simulink model "FluxObserver"  (R2026b)
settings: Solver=VariableStepAuto
undefined symbols (not defined in the file or in its folder): fluxCfg, pllCfg
libraries: AngleTracking x1
settings Model: Creator=24322  LastModifiedBy=24322

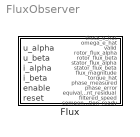
== system FluxObserver ==
  Flux : Subsystem  mask{cfg=fluxCfg, trackerCfg=pllCfg}
      mask prompts: cfg "Flux configuration"; trackerCfg "PLL configuration"

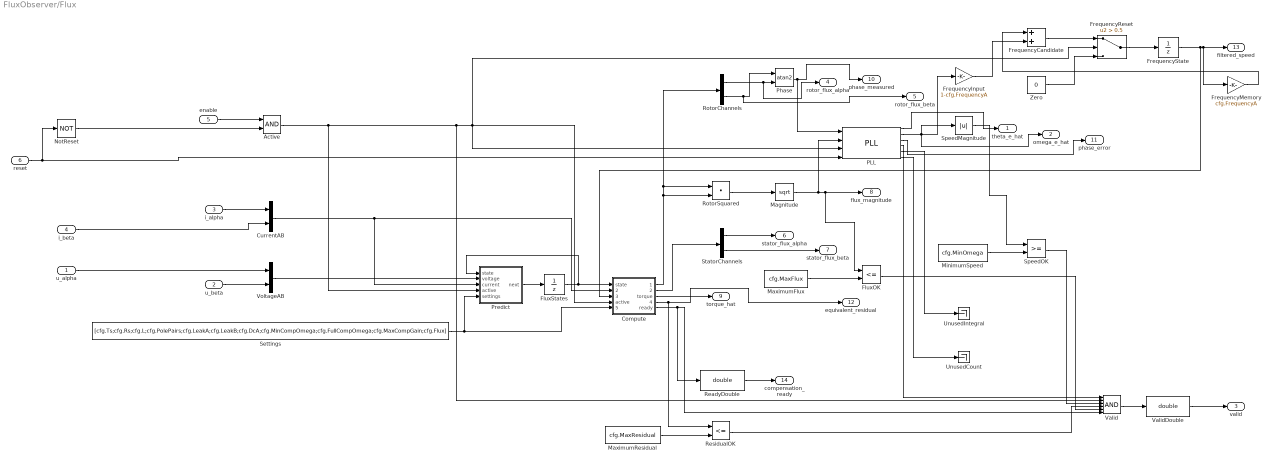
== system FluxObserver/Flux ==
  u_alpha : Inport  SampleTime=cfg.Ts
  u_beta : Inport  Port=2  SampleTime=cfg.Ts
  i_alpha : Inport  Port=3  SampleTime=cfg.Ts
  i_beta : Inport  Port=4  SampleTime=cfg.Ts
  enable : Inport  Port=5  SampleTime=cfg.Ts
  reset : Inport  Port=6  SampleTime=cfg.Ts
  Active : Logic  IconShape=distinctive  AllPortsSameDT=off  OutDataTypeStr=boolean
  Compute : MATLAB Function  TreatAsAtomicUnit=on
  CurrentAB : Mux  Inputs=2
  FluxOK : RelationalOperator  Operator=<=  OutDataTypeStr=boolean  RndMeth=Simplest  InputSameDT=off
  FluxStates : UnitDelay  InitialCondition=zeros(4,1)  SampleTime=cfg.Ts
  FrequencyCandidate : Sum
  FrequencyInput : Gain  Gain=1-cfg.FrequencyA
  FrequencyMemory : Gain  Gain=cfg.FrequencyA
  FrequencyReset : Switch  Criteria=u2 > Threshold  Threshold=0.5  SaturateOnIntegerOverflow=off  InputSameDT=off
  FrequencyState : UnitDelay  SampleTime=cfg.Ts
  Magnitude : Sqrt
  MaximumFlux : Constant  Value=cfg.MaxFlux
  MaximumResidual : Constant  Value=cfg.MaxResidual
  MinimumSpeed : Constant  Value=cfg.MinOmega
  NotReset : Logic  Operator=NOT  IconShape=distinctive  AllPortsSameDT=off  OutDataTypeStr=boolean
  PLL : AngleTracking/PLL  pllCfg=trackerCfg
  Phase : Trigonometry  Operator=atan2
  Predict : MATLAB Function  TreatAsAtomicUnit=on
  ReadyDouble : DataTypeConversion  OutDataTypeStr=double  SaturateOnIntegerOverflow=off  RndMeth=Floor
  ResidualOK : RelationalOperator  Operator=<=  OutDataTypeStr=boolean  RndMeth=Simplest  InputSameDT=off
  RotorChannels : Demux  Outputs=2
  RotorSquared : DotProduct  OutDataTypeStr=Inherit: Inherit via internal rule
  Settings : Constant  Value=[cfg.Ts;cfg.Rs;cfg.L;cfg.PolePairs;cfg.LeakA;cfg.LeakB;cfg.DcA;cfg.MinCompOmega;cfg.FullCompOmega;cfg.MaxCompGain;cfg.Flux]
  SpeedMagnitude : Abs  SaturateOnIntegerOverflow=off
  SpeedOK : RelationalOperator  OutDataTypeStr=boolean  RndMeth=Simplest  InputSameDT=off
  StatorChannels : Demux  Outputs=2
  UnusedCount : Terminator
  UnusedIntegral : Terminator
  Valid : Logic  Inputs=6  IconShape=distinctive  AllPortsSameDT=off  OutDataTypeStr=boolean
  ValidDouble : DataTypeConversion  OutDataTypeStr=double  SaturateOnIntegerOverflow=off  RndMeth=Floor
  VoltageAB : Mux  Inputs=2
  Zero : Constant  Value=0
  theta_e_hat : Outport
  omega_e_hat : Outport  Port=2
  valid : Outport  Port=3
  rotor_flux_alpha : Outport  Port=4
  rotor_flux_beta : Outport  Port=5
  stator_flux_alpha : Outport  Port=6
  stator_flux_beta : Outport  Port=7
  flux_magnitude : Outport  Port=8
  torque_hat : Outport  Port=9
  phase_measured : Outport  Port=10
  phase_error : Outport  Port=11
  equivalent_residual : Outport  Port=12
  filtered_speed : Outport  Port=13
  compensation_ready : Outport  Port=14
  wires:
  StatorChannels/2 -> stator_flux_beta/1
  StatorChannels/1 -> stator_flux_alpha/1
  PLL/6 -> UnusedCount/1
  PLL/5 -> UnusedIntegral/1
  PLL/4 -> Valid/1
  PLL/3 -> phase_error/1
  PLL/2 -> SpeedMagnitude/1, omega_e_hat/1, FrequencyInput/1
  PLL/1 -> theta_e_hat/1
  RotorChannels/1 -> Phase/2, rotor_flux_alpha/1
  RotorChannels/2 -> Phase/1, rotor_flux_beta/1
  RotorSquared/1 -> Magnitude/1
  Compute/5(ready) -> ReadyDouble/1, Valid/6
  Compute/4(residual) -> equivalent_residual/1, ResidualOK/1
  Compute/3(torque) -> torque_hat/1
  Compute/2(statorFlux) -> StatorChannels/1
  Compute/1(rotorFlux) -> RotorChannels/1, RotorSquared/1, RotorSquared/2
  Phase/1 -> PLL/1, phase_measured/1
  ReadyDouble/1 -> compensation_ready/1
  ValidDouble/1 -> valid/1
  Valid/1 -> ValidDouble/1
  FluxOK/1 -> Valid/5
  ResidualOK/1 -> Valid/4
  SpeedOK/1 -> Valid/3
  MaximumResidual/1 -> ResidualOK/2
  MinimumSpeed/1 -> SpeedOK/2
  SpeedMagnitude/1 -> SpeedOK/1
  MaximumFlux/1 -> FluxOK/2
  Magnitude/1 -> FluxOK/1, flux_magnitude/1, PLL/2
  FrequencyReset/1 -> FrequencyState/1
  Zero/1 -> FrequencyReset/3
  FrequencyCandidate/1 -> FrequencyReset/1
  FrequencyInput/1 -> FrequencyCandidate/2
  FrequencyMemory/1 -> FrequencyCandidate/1
  Predict/1(next) -> FluxStates/1
  VoltageAB/1 -> Predict/2(voltage)
  Settings/1 -> Compute/5(settings), Predict/5(settings)
  Active/1 -> PLL/3, Compute/4(active), FrequencyReset/2, Valid/2, Predict/4(active)
  FrequencyState/1 -> FrequencyMemory/1, filtered_speed/1, Compute/3(omega)
  CurrentAB/1 -> Compute/2(current), Predict/3(current)
  FluxStates/1 -> Compute/1(state), Predict/1(state)
  enable/1 -> Active/1
  NotReset/1 -> Active/2
  reset/1 -> PLL/4, NotReset/1
  i_beta/1 -> CurrentAB/2
  i_alpha/1 -> CurrentAB/1
  u_beta/1 -> VoltageAB/2
  u_alpha/1 -> VoltageAB/1

== matlab function FluxObserver/Flux/Predict ==
  data: state input; next output; voltage input; current input; active input; settings input
function next=flux_predict(state,voltage,current,active,settings)
%FLUX_PREDICT Leaky stator-flux integration and DC washout next states.
% state=[leaky_flux_ab;dc_flux_ab], each pair in Wb.
% settings=[Ts;Rs;L;p;LeakA;LeakB;DcA;MinCompOmega;FullCompOmega;MaxCompGain;Flux].
%#codegen
next=zeros(4,1,'like',state);
if ~active,return;end
z=state(1:2);dc=state(3:4);
next(1:2)=settings(5)*z+settings(6)*(voltage-settings(2)*current);
next(3:4)=settings(7)*dc+(1-settings(7))*z;
end

== matlab function FluxObserver/Flux/Compute ==
  data: state input; rotorFlux output; current input; omega input; active input; settings input; statorFlux output; torque output; residual output; ready output
function [rotorFlux,statorFlux,torque,residual,ready]=flux_compute(state,current,omega,active,settings)
%FLUX_COMPUTE Causal frequency-compensated SPMSM rotor flux from saved states.
% omega is a separate filtered PREVIOUS estimate, not the current PLL output.
% No voltage feedthrough, true angle, true speed or rotation-direction input.
%#codegen
rotorFlux=zeros(2,1,'like',state);statorFlux=zeros(2,1,'like',state);
torque=zeros(1,'like',state);residual=zeros(1,'like',state);ready=zeros(1,'like',state);
if ~active,return;end
filtered=state(1:2)-state(3:4);
coefficient=complex(ones(1,'like',state),zeros(1,'like',state));
if abs(omega)>settings(8)
    weight=min(1,(abs(omega)-settings(8))/(settings(9)-settings(8)));
    angle=omega*settings(1);unit=complex(cos(angle),sin(angle));
    raw=(unit-settings(5))*(unit-settings(7))/ ...
        (complex(omega*0,omega*settings(6))*(unit-1));
    gain=abs(raw);limited=gain>settings(10);
    if limited,raw=raw*(settings(10)/gain);end
    coefficient=1+weight*(raw-1);ready=cast(weight>=0.99 && ~limited,'like',state);
end
statorFlux=real(coefficient)*filtered+imag(coefficient)*[-filtered(2);filtered(1)];
rotorFlux=statorFlux-settings(3)*current;
torque=1.5*settings(4)*(rotorFlux(1)*current(2)-rotorFlux(2)*current(1));
residual=abs(hypot(rotorFlux(1),rotorFlux(2))-settings(11))/settings(3);
end
